simulink subsystem "Kep2Car"  (R2024b)
settings: Solver=VariableStepAuto  StartTime=0.0  StopTime=10.0  RelTol=1e-3
settings Model: Creator=marco  LastModifiedBy=domac

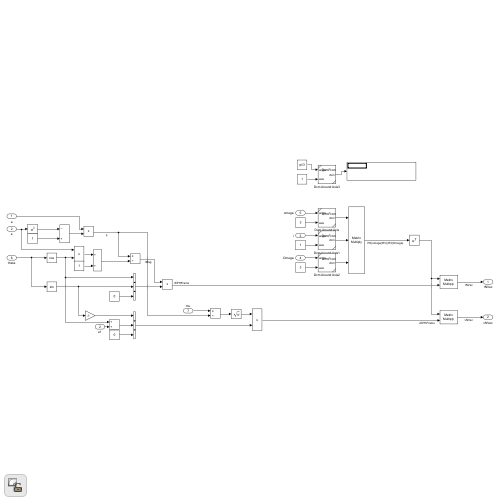
[thumbnail: Simulink's stored preview of the top-level diagram]
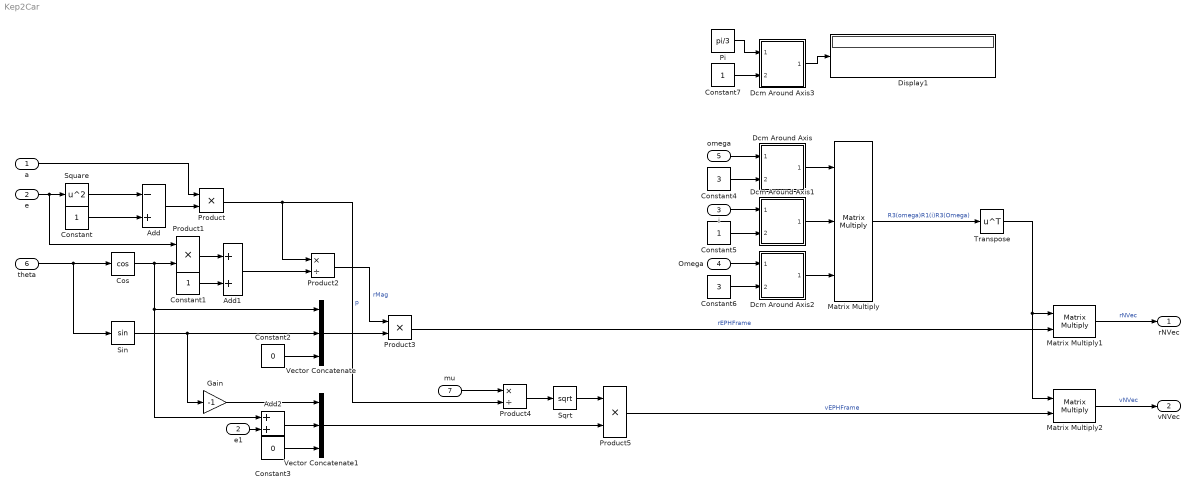
== system Kep2Car ==
  a : Inport
  e : Inport  Port=2
  i : Inport  Port=3
  Omega : Inport  Port=4
  omega : Inport  Port=5
  theta : Inport  Port=6
  mu : Inport  Port=7
  Add : Sum  Inputs=-+
  Add1 : Sum
  Add2 : Sum
  Constant : Constant
  Constant1 : Constant
  Constant2 : Constant  Value=0
  Constant3 : Constant  Value=0
  Constant4 : Constant  Value=3  OutDataTypeStr=Inherit: Inherit via back propagation
  Constant5 : Constant  OutDataTypeStr=Inherit: Inherit via back propagation
  Constant6 : Constant  Value=3  OutDataTypeStr=Inherit: Inherit via back propagation
  Constant7 : Constant
  Cos : Trigonometry  Operator=cos
  Dcm Around Axis{,1..3} (4 alike) : Subsystem  ReferencedSubsystem=DcmFromAxis
  Display1 : Display
  Gain : Gain  Gain=-1
  Matrix Multiply : Product  Inputs=3  Multiplication=Matrix(*)
  Matrix Multiply1 : Product  Multiplication=Matrix(*)
  Matrix Multiply2 : Product  Multiplication=Matrix(*)
  Pi : Constant  Value=pi/3  OutDataTypeStr=Inherit: Inherit via back propagation
  Product{,1,3,5} (4 alike) : Product
  Product2 : Product  Inputs=*/
  Product4 : Product  Inputs=*/
  Sin : Trigonometry
  Sqrt : Sqrt
  Square : Math  Operator=square
  Transpose : Math  Operator=transpose
  Vector Concatenate : Concatenate  NumInputs=3
  Vector Concatenate1 : Concatenate  NumInputs=3
  e1 : InportShadow  Port=2
  rNVec : Outport  PortDimensions=[3, 1]
  vNVec : Outport  Port=2  PortDimensions=[3, 1]
  wires:
  e/1 -> Square/1, Product1/1
  Square/1 -> Add/1
  Constant/1 -> Add/2
  Add/1 -> Product/2
  a/1 -> Product/1
  Product/1 -> Product2/1, Product4/2  "p"
  theta/1 -> Cos/1, Sin/1
  Cos/1 -> Product1/2, Add2/1, Vector Concatenate/1
  Product1/1 -> Add1/1
  Constant1/1 -> Add1/2
  Add1/1 -> Product2/2
  Product2/1 -> Product3/1  "rMag"
  Sin/1 -> Vector Concatenate/2, Gain/1
  Constant2/1 -> Vector Concatenate/3
  Vector Concatenate/1 -> Product3/2
  Product3/1 -> Matrix Multiply1/2  "rEPHFrame"
  e1/1 -> Add2/2
  Add2/1 -> Vector Concatenate1/2
  Constant3/1 -> Vector Concatenate1/3
  Vector Concatenate1/1 -> Product5/2
  mu/1 -> Product4/1
  Product4/1 -> Sqrt/1
  Sqrt/1 -> Product5/1
  Product5/1 -> Matrix Multiply2/2  "vEPHFrame"
  Matrix Multiply/1 -> Transpose/1  "R3(omega)R1(i)R3(Omega)"
  Matrix Multiply1/1 -> rNVec/1  "rNVec"
  Matrix Multiply2/1 -> vNVec/1  "vNVec"
  Transpose/1 -> Matrix Multiply1/1, Matrix Multiply2/1
  Constant4/1 -> Dcm Around Axis/2
  omega/1 -> Dcm Around Axis/1
  Constant6/1 -> Dcm Around Axis2/2
  Omega/1 -> Dcm Around Axis2/1
  i/1 -> Dcm Around Axis1/1
  Constant5/1 -> Dcm Around Axis1/2
  Dcm Around Axis/1 -> Matrix Multiply/1
  Dcm Around Axis1/1 -> Matrix Multiply/2
  Dcm Around Axis2/1 -> Matrix Multiply/3
  Gain/1 -> Vector Concatenate1/1
  Constant7/1 -> Dcm Around Axis3/2
  Pi/1 -> Dcm Around Axis3/1
  Dcm Around Axis3/1 -> Display1/1
